simulink model "xz_packaging_automatic"  (R2025b)
settings: Solver=ode15s  StartTime=0.0  StopTime=13.05  MaxStep=0.001  RelTol=1e-6  AbsTol=1e-9
model workspace: external: MATLAB File xz_packaging_automatic_DataFile.m (data not in the file)
values from neighbouring files (symbols this model uses):
  payloadMass_kg = 0.25    [xz_packaging_automatic_DataFile.m]
undefined symbols (not defined in the file or in its folder): smiData, X, Y, Z
libraries: sm_lib x2549, nesl_utility x31
(part 38 of 38)

== matlab function xz_packaging_automatic/Bench trajectory reference ==
  data: t input; x output; stage input; start input; z output; cycle input; holdPose input; owner input; belts output; cartonY output; carrierY output
function [x,z,belts,cartonY,carrierY] = automatic_reference(t,stage,start,cycle,holdPose,owner)
% Rows are position (m), velocity (m/s), acceleration (m/s^2).
% X travel is positive world X. Tool Z travel is positive down.
dt = t-start;
x = [0.05;0;0];
z = [0.1755;0;0];
switch stage
    case {0,20,21}
        z(1) = 0.024;
    case 1
        if dt < 1
            z = stroke(dt,1,0.024,0.1705);
        else
            z = stroke(dt-1,1.15,0.1705,0.1755);
        end
    case 3
        z = stroke(dt,0.30,0.1755,0.174);
    case 4
        z = stroke(dt,1,0.174,0.024);
    case 5
        z(1) = 0.024;
        x = stroke(dt,1.30,0.05,0.45);
    case 6
        x(1) = 0.45;
        if dt < 1
            z = stroke(dt,1,0.024,0.1705);
        else
            z = stroke(dt-1,0.80,0.1705,0.174);
        end
    case 7
        x(1) = 0.45;
        z = stroke(dt,0.40,0.174,0.1755);
    case {8,14}
        x(1) = 0.45;
    case {9,12}
        if stage == 9
            x(1) = 0.45;
        end
        if dt < 0.30
            z = stroke(dt,0.30,0.1755,0.174);
        else
            z = stroke(dt-0.30,1,0.174,0.024);
        end
    case {22,24}
        x(1) = 0.45;
        z(1) = 0.024;
    case 23
        x = stroke(dt,1.30,0.45,0.05);
        z(1) = 0.024;
    case 13
        z(1) = 0.024;
    case 90
        x(1) = holdPose(1);
        z(1) = holdPose(2);
end
base = cycle(4:5);
in = [base(1);0;0];
out = [base(2);0;0];
if stage==21
    in = stroke(dt,1,base(1),base(1)+0.16*cycle(7));
    out = stroke(dt,1,base(2),base(2)+0.015*cycle(8));
elseif any(stage==[1:9 11:13 22:24])
    in(1) = base(1)+0.16;
    out(1) = base(2)+0.015;
    if stage==22
        out = stroke(dt,1,out(1),out(1)+0.16*cycle(8));
    elseif stage==23 || stage==24
        out(1) = out(1)+0.16;
    end
elseif stage==90
    in(1) = holdPose(3);
    out(1) = holdPose(4);
end
belts = [in;out];
carrierY = out-[base(2)+0.015;0;0];
if stage==20 && cycle(9)>0.5
    carrierY = [0.16;0;0];
end
cartonY = [base(1)+0.16;0;0]-in;
if owner==2
    cartonY = zeros(3,1);
elseif owner==3
    cartonY = carrierY;
end

end

function y = stroke(t,duration,first,last)
s = min(1,max(0,t/duration));
d = last-first;
y = [first+d*s^3*(10-15*s+6*s^2); ...
     d/duration*30*s^2*(1-s)^2; ...
     d/duration^2*60*s*(1-s)*(1-2*s)];
end

== matlab function xz_packaging_automatic/Carton coupling ==
  data: owner input; cx output; q input; v input; a input; process input; cz output; load output; required output; contact output; payload input
function [cx,cz,load,required,contact] = carton_coupling(owner,q,v,a,process,payload)
% The carton is constrained to the tool only while carried.
cx = zeros(3,1);
cz = zeros(3,1);
load = zeros(3,1);
required = 0;
contact = double((owner==1 && process(1)>0.5 && abs(q(1)-0.05)<0.0005) || ...
    (owner==3 && process(2)>0.5 && abs(process(3))<=0.0005 && abs(q(1)-0.45)<0.0005));
if owner==2
    cx = [q(1)-0.05;v(1);a(1)];
    cz = [max(0,0.174-q(2));-v(2);-a(2)];
    load = payload*[a(1);0;9.80665-a(2)];
    moment = abs(load(1))*0.015+load(3)*0.002;
    required = 2*(load(3)/2+moment/0.036+abs(load(1))/(2*0.30));
elseif owner==3
    cx(1) = 0.4;
end
end
